simulink model "wattcredit_hw_fast"  (R2023a)
settings: Solver=FixedStepDiscrete  StartTime=0.0  StopTime=0.3  FixedStep=Tp  RelTol=1e-3
undefined symbols (not defined in the file or in its folder): f0, hw, Tp, Ts, Vnom
libraries: spsSeriesRLCBranchLib x5, spsDiodeLib x4, spsCurrentMeasurementLib x2, spsACVoltageSourceLib x2, spsIdealSwitchLib x1, spspowerguiLib x1
settings Model: Creator=ruthm  LastModifiedBy=ruthm

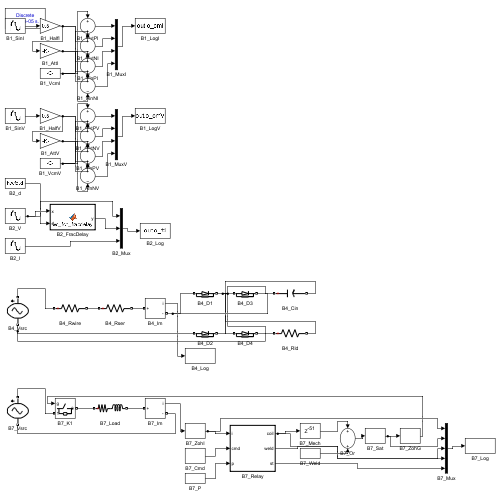
[thumbnail: Simulink's stored preview of the top-level diagram]
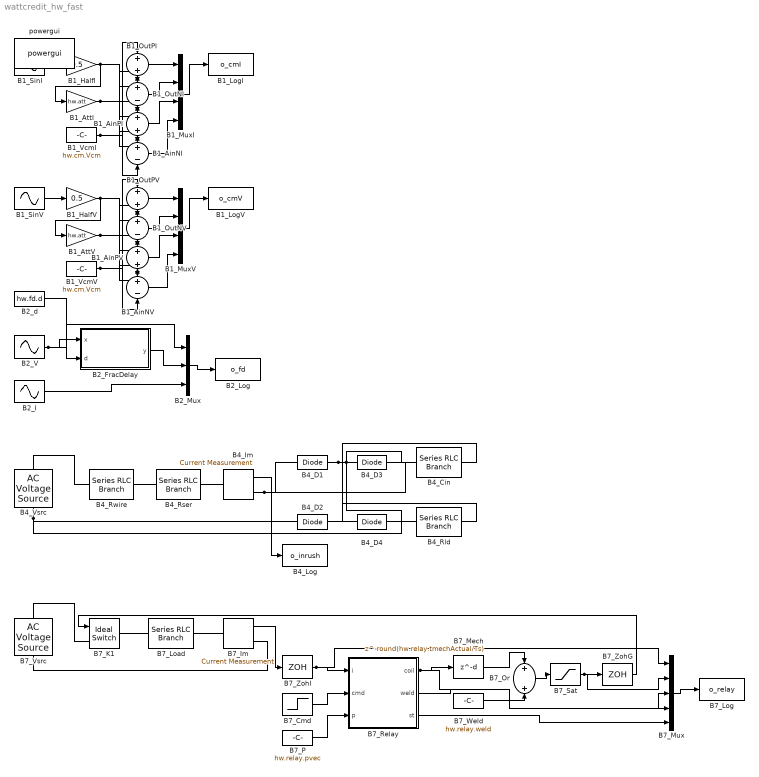
== system wattcredit_hw_fast ==
  B1_AinNI : Sum  Inputs=+-
  B1_AinNV : Sum  Inputs=+-
  B1_AinPI : Sum
  B1_AinPV : Sum
  B1_AttI : Gain  Gain=hw.att
  B1_AttV : Gain  Gain=hw.att
  B1_HalfI : Gain  Gain=0.5
  B1_HalfV : Gain  Gain=0.5
  B1_LogI : ToWorkspace  VariableName=o_cmI  SampleTime=-1
  B1_LogV : ToWorkspace  VariableName=o_cmV  SampleTime=-1
  B1_MuxI : Mux
  B1_MuxV : Mux
  B1_OutNI : Sum  Inputs=+-
  B1_OutNV : Sum  Inputs=+-
  B1_OutPI : Sum
  B1_OutPV : Sum
  B1_SinI : Sin  Amplitude=hw.cm.vdI  Frequency=2*pi*f0  SampleTime=Ts
  B1_SinV : Sin  Amplitude=hw.cm.vdV  Frequency=2*pi*f0  SampleTime=Ts
  B1_VcmI : Constant  Value=hw.cm.Vcm
  B1_VcmV : Constant  Value=hw.cm.Vcm
  B2_FracDelay : MATLAB Function  TreatAsAtomicUnit=on
  B2_I : Sin  Amplitude=14.14  Frequency=2*pi*f0  Phase=-pi/3  SampleTime=Ts
  B2_Log : ToWorkspace  VariableName=o_fd  SampleTime=-1
  B2_Mux : Mux  Inputs=3
  B2_V : Sin  Amplitude=325  Frequency=2*pi*f0  SampleTime=Ts
  B2_d : Constant  Value=hw.fd.d
  B4_Cin : spsSeriesRLCBranchLib/Series RLC Branch  LConnTagsString=__new0  RConnTagsString=__new0  BranchType=C  Resistance=1  Inductance=1e-3  SetiL0=off  InitialCurrent=0  Capacitance=hw.inrush.Cin  Setx0=off  InitialVoltage=0  Measurements=None
  B4_D{1..4} (4 alike) : spsDiodeLib/Diode  Ron=0.05  Lon=0  Vf=0.8  IC=0  UseSnubber=0  Rs=500  Cs=250e-9  Measurements=off
  B4_Im : spsCurrentMeasurementLib/Current Measurement  PhasorSimulation=off  OutputType=Complex  PSBequivalent=0
  B4_Log : ToWorkspace  VariableName=o_inrush  SampleTime=-1
  B4_Rld : spsSeriesRLCBranchLib/Series RLC Branch  LConnTagsString=__new0  RConnTagsString=__new0  BranchType=R  Resistance=hw.inrush.Rld  Inductance=1e-3  SetiL0=off  InitialCurrent=0  Capacitance=1e-6  Setx0=off  InitialVoltage=0  Measurements=None
  B4_Rser : spsSeriesRLCBranchLib/Series RLC Branch  LConnTagsString=__new0  RConnTagsString=__new0  BranchType=R  Resistance=max(hw.inrush.Rser,1e-3)  Inductance=1e-3  SetiL0=off  InitialCurrent=0  Capacitance=1e-6  Setx0=off  InitialVoltage=0  Measurements=None
  B4_Rwire : spsSeriesRLCBranchLib/Series RLC Branch  LConnTagsString=__new0  RConnTagsString=__new0  BranchType=R  Resistance=hw.inrush.Rwire  Inductance=1e-3  SetiL0=off  InitialCurrent=0  Capacitance=1e-6  Setx0=off  InitialVoltage=0  Measurements=None
  B4_Vsrc : spsACVoltageSourceLib/AC Voltage Source  Amplitude=hw.inrush.Vpk  Phase=90  Frequency=f0  SampleTime=0  Measurements=None  BusType=swing  Pref=10e3  Qref=0  Qmin=-inf  Qmax=+inf
  B7_Cmd : Step  Time=hw.relay.tcmd  Before=1  After=0  SampleTime=Ts
  B7_Im : spsCurrentMeasurementLib/Current Measurement  PhasorSimulation=off  OutputType=Complex  PSBequivalent=0
  B7_K1 : spsIdealSwitchLib/Ideal Switch  Ron=1e-3  Lon=0  IC=0  Rs=1e6  Cs=inf  Measurements=off
  B7_Load : spsSeriesRLCBranchLib/Series RLC Branch  LConnTagsString=__new0  RConnTagsString=__new0  BranchType=RL  Resistance=hw.relay.R  Inductance=hw.relay.L  SetiL0=off  InitialCurrent=0  Capacitance=1e-6  Setx0=off  InitialVoltage=0  Measurements=None
  B7_Log : ToWorkspace  VariableName=o_relay  SampleTime=-1
  B7_Mech : Delay  DelayLength=round(hw.relay.tmechActual/Ts)  InitialCondition=1  SampleTime=Ts
  B7_Mux : Mux  Inputs=5
  B7_Or : Sum
  B7_P : Constant  Value=hw.relay.pvec
  B7_Relay : MATLAB Function  TreatAsAtomicUnit=on
  B7_Sat : Saturate  UpperLimit=1  LowerLimit=0
  B7_Vsrc : spsACVoltageSourceLib/AC Voltage Source  Amplitude=Vnom*sqrt(2)  Phase=0  Frequency=f0  SampleTime=0  Measurements=None  BusType=swing  Pref=10e3  Qref=0  Qmin=-inf  Qmax=+inf
  B7_Weld : Constant  Value=hw.relay.weld
  B7_ZohG : ZeroOrderHold  SampleTime=Tp
  B7_ZohI : ZeroOrderHold  SampleTime=Ts
  powergui : spspowerguiLib/powergui  Priority=1  SimulationMode=Discrete  SampleTime=Tp  frequency=60  Iterations=50  frequencyindice=60  Pbase=100e6  ErrMax=1e-4  UnitsV=kV  UnitsW=MW  buscounter=0  FunctionMessages=off  echomessages=off  EnableUseOfTLC=off  CurrentSourceSwitches=off  DisableSnubberDevices=off  DisableRonSwitches=off  DisableVfSwitches=off  DisplayEquations=off  AutomaticDiscreteSolvers=off  SolverType=Tustin/Backward Euler (TBE)  Interpol=off  ExternalGateDelay=off  methode=off  Ts=100  x0status=blocks  SPID=on  SwTol=0  HookPort=off  NonlinearTolerance=1e-4  nMaxIteration=100  ContinueOnMaxIteration=off  RestoreLinks=warning  ResistiveCurrentMeasurement=off  Frange=[0:2:500]  Ylog=off  Xlog=on  ShowGrid=off  save=off  variable=ZData  structure=0  ZoomFFT=off  StartTime=0.0  cycles=1  DisplayStyle=1  fundamental=60  FreqAxis=off  MaxFrequency=1000  frequencyindicesteady=1  RmsSteady=1  display=off
  wires:
  B1_SinI/1 -> B1_HalfI/1
  B1_HalfI/1 -> B1_OutPI/2, B1_OutNI/2, B1_AttI/1
  B1_VcmI/1 -> B1_OutPI/1, B1_OutNI/1, B1_AinPI/1, B1_AinNI/1
  B1_AttI/1 -> B1_AinPI/2, B1_AinNI/2
  B1_OutPI/1 -> B1_MuxI/1
  B1_OutNI/1 -> B1_MuxI/2
  B1_AinPI/1 -> B1_MuxI/3
  B1_AinNI/1 -> B1_MuxI/4
  B1_MuxI/1 -> B1_LogI/1
  B1_SinV/1 -> B1_HalfV/1
  B1_HalfV/1 -> B1_OutPV/2, B1_OutNV/2, B1_AttV/1
  B1_VcmV/1 -> B1_OutPV/1, B1_OutNV/1, B1_AinPV/1, B1_AinNV/1
  B1_AttV/1 -> B1_AinPV/2, B1_AinNV/2
  B1_OutPV/1 -> B1_MuxV/1
  B1_OutNV/1 -> B1_MuxV/2
  B1_AinPV/1 -> B1_MuxV/3
  B1_AinNV/1 -> B1_MuxV/4
  B1_MuxV/1 -> B1_LogV/1
  B2_V/1 -> B2_FracDelay/1(x), B2_Mux/1
  B2_d/1 -> B2_FracDelay/2(d)
  B2_FracDelay/1(y) -> B2_Mux/2
  B2_I/1 -> B2_Mux/3
  B2_Mux/1 -> B2_Log/1
  B4_Im/1 -> B4_Log/1
  B7_Im/1 -> B7_ZohI/1
  B7_ZohI/1 -> B7_Relay/1(i), B7_Mux/1
  B7_Cmd/1 -> B7_Relay/2(cmd)
  B7_P/1 -> B7_Relay/3(p)
  B7_Relay/1(coil) -> B7_Mech/1, B7_Mux/3
  B7_Mech/1 -> B7_Or/1
  B7_Weld/1 -> B7_Or/2
  B7_Or/1 -> B7_Sat/1
  B7_Sat/1 -> B7_ZohG/1, B7_Mux/2
  B7_ZohG/1 -> B7_K1/1
  B7_Relay/2(weld) -> B7_Mux/4
  B7_Relay/3(st) -> B7_Mux/5
  B7_Mux/1 -> B7_Log/1
  connections:
  B4_Vsrc/RConn1 -- B4_Rwire/LConn1
  B4_Rwire/RConn1 -- B4_Rser/LConn1
  B4_Rser/RConn1 -- B4_Im/LConn1
  B4_D1/LConn1 -- B4_Im/RConn1 -- B4_D3/RConn1
  B4_D2/LConn1 -- B4_Vsrc/LConn1 -- B4_D4/RConn1
  B4_D2/RConn1 -- B4_D1/RConn1 -- B4_Cin/LConn1 -- B4_Rld/LConn1
  B4_D4/LConn1 -- B4_D3/LConn1 -- B4_Cin/RConn1 -- B4_Rld/RConn1
  B7_Vsrc/RConn1 -- B7_K1/LConn1
  B7_K1/RConn1 -- B7_Load/LConn1
  B7_Load/RConn1 -- B7_Im/LConn1
  B7_Im/RConn1 -- B7_Vsrc/LConn1

== matlab function wattcredit_hw_fast/B7_Relay ==
  data: i input; coil output; cmd input; p input; weld output; st output
function [coil, weld, st] = wc_fcn_relay(i, cmd, p)
%WC_FCN_RELAY  Relay controller (paste into a MATLAB Function block). One call per sample.
%  i    : current sample (A)               cmd : 1 = keep closed, 0 = open
%  p    : [fs f0 tmech tweld iweld]        tmech = coil-off to contact-part time (s)
%  coil : 1 = energised (closed)           weld : latched 1 if current persists tweld after the open command
%  st   : 0 idle, 1 waiting for current zero, 2 timing, 3 coil released, 4 weld check done
%  Opening is keyed on the CURRENT zero crossing (not the grid zero crossing: for an inductive load the
%  current zero lags the voltage zero by phi/w). The coil is released so the contacts part tmech later, on a
%  following current zero: wait = (T/2 - mod(tmech, T/2)) mod T/2.
persistent state prev cmdPrev nWait nSince win k coilS weldS
spc = round(p(1)/p(2));
if isempty(state)
    state = 0; prev = 0; cmdPrev = 1; nWait = 0; nSince = 0; win = zeros(1, 256); k = 0; coilS = 1; weldS = 0;
end
k = mod(k, spc) + 1;
win(k) = i*i;
irms = sqrt(sum(win(1:spc))/spc);                 % one-cycle sliding RMS
zc = (prev <= 0 && i > 0) || (prev >= 0 && i < 0);
prev = i;
if cmd == 0 && cmdPrev == 1 && state == 0
    state = 1; nSince = 0;                        % open command received: wait for a current zero
end
if cmd == 1 && state == 1
    state = 0;                                    % command withdrawn before the coil was released
end
if cmd == 1 && cmdPrev == 0 && state >= 3 && weldS == 0
    coilS = 1; state = 0;                         % re-close (only if no weld is latched)
end
cmdPrev = cmd;
if state >= 1
    nSince = nSince + 1;
end
th = 0.5/p(2);
if state == 1 && zc
    nWait = round(mod(th - mod(p(3), th), th)*p(1));
    state = 2;
end
if state == 2
    if nWait <= 0
        coilS = 0; state = 3;
    else
        nWait = nWait - 1;
    end
end
if state == 3 && nSince >= round(p(4)*p(1))
    if irms >= p(5), weldS = 1; end
    state = 4;
end
coil = coilS;
weld = weldS;
st = state;
end

== matlab function wattcredit_hw_fast/B2_FracDelay ==
  data: x input; y output; d input
function y = wc_fcn_fracdelay(x, d)
%WC_FCN_FRACDELAY  Fractional-sample delay by linear interpolation (paste into a MATLAB Function block).
%  y[n] = (1-d)*x[n] + d*x[n-1],  0 <= d < 1.  Delays the stream by d samples: a phase lag of 2*pi*f0*d/fs at f0.
%  Put it in the path of the channel that LEADS (usually voltage, because the current channel has the slower filter
%  or the inductive shunt), with d set at calibration from the measured phase error. Gain error is below 0.03 % at 50 Hz for d <= 0.36.
persistent xp
if isempty(xp), xp = 0; end
y = (1 - d)*x + d*xp;
xp = x;
end
